simulink library "SNS_Library"  (R2025b)
settings: Solver=VariableStepAuto  StartTime=0.0  StopTime=10.0  RelTol=1e-3
libraries: simulink x3
settings Model: Creator=Ben Bolen  LastModifiedBy=Ben

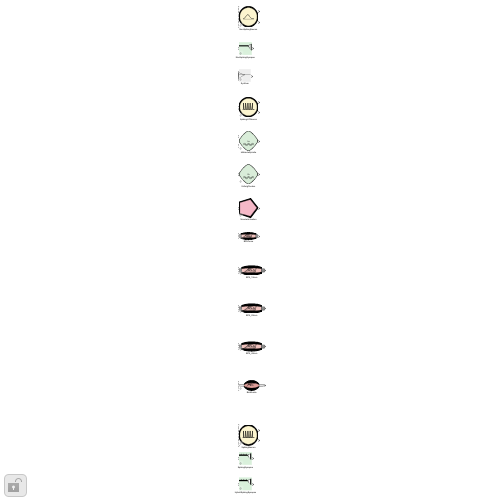
[thumbnail: Simulink's stored preview of the top-level diagram]
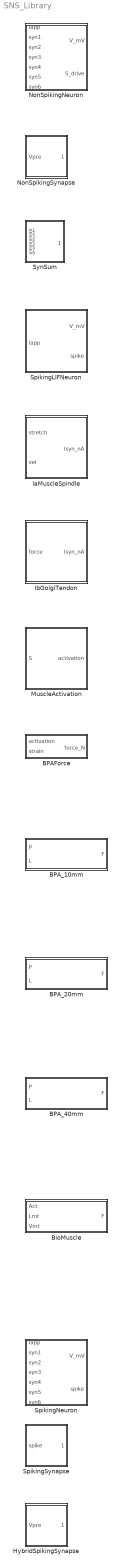
== system SNS_Library ==
  BPAForce : Subsystem  mask(SNS BPA Force Element){Fmax=500, epsMax=0.25}
      mask prompts: Fmax "Max isometric force Fmax (N)"; epsMax "Max contraction strain epsMax (0..1)"
      mask help: Simple BPA (pneumatic artificial muscle) force: F = Fmax*A*max(0, epsMax - strain). Replace with MonoPam/Xi-corrected prediction when available.
      mask Display:
      | patch([-0.7 -0.6708 -0.6417 -0.6125 -0.5833 -0.5542 -0.525 -0.4958 -0.4667 -0.4375 -0.4083 -0.3792 -0.35 -0.3208 -0.2917 -0.2625 -0.2333 -0.2042 -0.175 -0.1458 -0.1167 -0.0875 -0.05833 -0.02917 0 0.02917 0.05833 0.0875 0.1167 0.1458 0.175 0.2042 0.2333 0.2625 0.2917 0.3208 0.35 0.3792 0.4083 0.4375 0.4667 0.4958 0.525 0.5542 0.5833 0.6125 0.6417 0.6708 0.7 0.7 0.6708 0.6417 0.6125 0.5833 0.5542 0.525 0.4958 0.4667 0.4375 0.4083 0.3792 0.35 0.3208 0.2917 0.2625 0.2333 0.2042 0.175 0.1458 0.1167 0.0875 0.05833 0.02917 0 -0.02917 -0.05833 -0.0875 -0.1167 -0.1458 -0.175 -0.2042 -0.2333 -0.2625 -0.2917 -0.3208 -0.35 -0.3792 -0.4083 -0.4375 -0.4667 -0.4958 -0.525 -0.5542 -0.5833 -0.6125 -0.6417 -0.6708 -0.7], [0.395 0.4138 0.4317 0.4489 0.4653 0.4809 0.4956 0.5096 0.5228 0.5352 0.5467 0.5575 0.5675 0.5767 0.5851 0.5927 0.5994 0.6054 0.6106 0.615 0.6186 0.6214 0.6234 0.6246 0.625 0.6246 0.6234 0.6214 0.6186 0.615 0.6106 0.6054 0.5994 0.5927 0.5851 0.5767 0.5675 0.5575 0.5467 0.5352 0.5228 0.5096 0.4956 0.4809 0.4653 0.4489 0.4317 0.4138 0.395 -0.395 -0.4138 -0.4317 -0.4489 -0.4653 -0.4809 -0.4956 -0.5096 -0.5228 -0.5352 -0.5467 -0.5575 -0.5675 -0.5767 -0.5851 -0.5927 -0.5994 -0.6054 -0.6106 -0.615 -0.6186 -0.6214 -0.6234 -0.6246 -0.625 -0.6246 -0.6234 -0.6214 -0.6186 -0.615 -0.6106 -0.6054 -0.5994 -0.5927 -0.5851 -0.5767 -0.5675 -0.5575 -0.5467 -0.5352 -0.5228 -0.5096 -0.4956 -0.4809 -0.4653 -0.4489 -0.4317 -0.4138 -0.395], [0 0 0]);
      | patch([-0.7 -0.6708 -0.6417 -0.6125 -0.5833 -0.5542 -0.525 -0.4958 -0.4667 -0.4375 -0.4083 -0.3792 -0.35 -0.3208 -0.2917 -0.2625 -0.2333 -0.2042 -0.175 -0.1458 -0.1167 -0.0875 -0.05833 -0.02917 0 0.02917 0.05833 0.0875 0.1167 0.1458 0.175 0.2042 0.2333 0.2625 0.2917 0.3208 0.35 0.3792 0.4083 0.4375 0.4667 0.4958 0.525 0.5542 0.5833 0.6125 0.6417 0.6708 0.7 0.7 0.6708 0.6417 0.6125 0.5833 0.5542 0.525 0.4958 0.4667 0.4375 0.4083 0.3792 0.35 0.3208 0.2917 0.2625 0.2333 0.2042 0.175 0.1458 0.1167 0.0875 0.05833 0.02917 0 -0.02917 -0.05833 -0.0875 -0.1167 -0.1458 -0.175 -0.2042 -0.2333 -0.2625 -0.2917 -0.3208 -0.35 -0.3792 -0.4083 -0.4375 -0.4667 -0.4958 -0.525 -0.5542 -0.5833 -0.6125 -0.6417 -0.6708 -0.7], [0.185 0.1944 0.2034 0.212 0.2201 0.2279 0.2353 0.2423 0.2489 0.2551 0.2609 0.2663 0.2712 0.2758 0.28 0.2838 0.2872 0.2902 0.2928 0.295 0.2968 0.2982 0.2992 0.2998 0.3 0.2998 0.2992 0.2982 0.2968 0.295 0.2928 0.2902 0.2872 0.2838 0.28 0.2758 0.2712 0.2663 0.2609 0.2551 0.2489 0.2423 0.2353 0.2279 0.2201 0.212 0.2034 0.1944 0.185 -0.185 -0.1944 -0.2034 -0.212 -0.2201 -0.2279 -0.2353 -0.2423 -0.2489 -0.2551 -0.2609 -0.2663 -0.2712 -0.2758 -0.28 -0.2838 -0.2872 -0.2902 -0.2928 -0.295 -0.2968 -0.2982 -0.2992 -0.2998 -0.3 -0.2998 -0.2992 -0.2982 -0.2968 -0.295 -0.2928 -0.2902 -0.2872 -0.2838 -0.28 -0.2758 -0.2712 -0.2663 -0.2609 -0.2551 -0.2489 -0.2423 -0.2353 -0.2279 -0.2201 -0.212 -0.2034 -0.1944 -0.185], [0.94 0.76 0.74]);
      | color('black');
      | plot([-0.64 -0.1835], [-0.34 0.2456]);
      | plot([-0.64 0.1835], [-0.34 -0.2456]);
      | plot([-0.465 -0.2243], [-0.165 0.2642]);
      | plot([-0.465 0.2243], [-0.165 -0.2642]);
      | plot([-0.29 -0.2522], [0.01 0.27]);
      | plot([-0.29 0.2522], [0.01 -0.27]);
      | plot([-0.115 -0.2672], [0.185 0.2628]);
      | plot([-0.115 0.2672], [0.185 -0.2628]);
      | plot([0.06 -0.2692], [0.36 0.2426]);
      | plot([0.06 0.2692], [0.36 -0.2426]);
      | plot([0.235 -0.2583], [0.535 0.2095]);
      | plot([0.235 0.2583], [0.535 -0.2095]);
      | plot([0.41 -0.2345], [0.66 0.178]);
      | plot([0.41 0.2345], [0.66 -0.178]);
      | patch([0.7 0.9 0.9 0.7], [-0.218 -0.218 0.218 0.218], [0 0 0]);
      | patch([0.7 0.9 0.9 0.7], [-0.2 -0.2 0.2 0.2], [0.55 0.55 0.55]);
      | patch([-0.7 -0.9 -0.9 -0.7], [-0.218 -0.218 0.218 0.218], [0 0 0]);
      | patch([-0.7 -0.9 -0.9 -0.7], [-0.2 -0.2 0.2 0.2], [0.55 0.55 0.55]);
      | disp('BPA');
  BPA_10mm : Subsystem  mask(SNS BPA 10 mm Actuator){Rest=0.20, Kmax=0.165, TendonL=0, FittingL=0}
      mask prompts: Rest "Resting length Rest (m)"; Kmax "Fully-contracted length Kmax (m)"; TendonL "Tendon length (m)"; FittingL "One end-fitting length (m)"
      mask help: Real Festo BPA actuator, 10 mm ID, Ben's equations: F = Fmax*[a0*(exp(-a1*rel)-1) + (P/620)*exp(-a3*rel^2)], rel = contraction/KMAX, contraction = (Rest-(L-TendonL-2*FittingL))/Rest. Zero force for rel>=1 and F<0 (festo4.m). Fmax = maxBPAforce(Rest,620) is baked into the internal gain (edit inside the block to override); Inputs: P [kPa], L [m]. Output: F [N].
      mask Display:
      | patch([-0.7 -0.6708 -0.6417 -0.6125 -0.5833 -0.5542 -0.525 -0.4958 -0.4667 -0.4375 -0.4083 -0.3792 -0.35 -0.3208 -0.2917 -0.2625 -0.2333 -0.2042 -0.175 -0.1458 -0.1167 -0.0875 -0.05833 -0.02917 0 0.02917 0.05833 0.0875 0.1167 0.1458 0.175 0.2042 0.2333 0.2625 0.2917 0.3208 0.35 0.3792 0.4083 0.4375 0.4667 0.4958 0.525 0.5542 0.5833 0.6125 0.6417 0.6708 0.7 0.7 0.6708 0.6417 0.6125 0.5833 0.5542 0.525 0.4958 0.4667 0.4375 0.4083 0.3792 0.35 0.3208 0.2917 0.2625 0.2333 0.2042 0.175 0.1458 0.1167 0.0875 0.05833 0.02917 0 -0.02917 -0.05833 -0.0875 -0.1167 -0.1458 -0.175 -0.2042 -0.2333 -0.2625 -0.2917 -0.3208 -0.35 -0.3792 -0.4083 -0.4375 -0.4667 -0.4958 -0.525 -0.5542 -0.5833 -0.6125 -0.6417 -0.6708 -0.7], [0.395 0.4138 0.4317 0.4489 0.4653 0.4809 0.4956 0.5096 0.5228 0.5352 0.5467 0.5575 0.5675 0.5767 0.5851 0.5927 0.5994 0.6054 0.6106 0.615 0.6186 0.6214 0.6234 0.6246 0.625 0.6246 0.6234 0.6214 0.6186 0.615 0.6106 0.6054 0.5994 0.5927 0.5851 0.5767 0.5675 0.5575 0.5467 0.5352 0.5228 0.5096 0.4956 0.4809 0.4653 0.4489 0.4317 0.4138 0.395 -0.395 -0.4138 -0.4317 -0.4489 -0.4653 -0.4809 -0.4956 -0.5096 -0.5228 -0.5352 -0.5467 -0.5575 -0.5675 -0.5767 -0.5851 -0.5927 -0.5994 -0.6054 -0.6106 -0.615 -0.6186 -0.6214 -0.6234 -0.6246 -0.625 -0.6246 -0.6234 -0.6214 -0.6186 -0.615 -0.6106 -0.6054 -0.5994 -0.5927 -0.5851 -0.5767 -0.5675 -0.5575 -0.5467 -0.5352 -0.5228 -0.5096 -0.4956 -0.4809 -0.4653 -0.4489 -0.4317 -0.4138 -0.395], [0 0 0]);
      | patch([-0.7 -0.6708 -0.6417 -0.6125 -0.5833 -0.5542 -0.525 -0.4958 -0.4667 -0.4375 -0.4083 -0.3792 -0.35 -0.3208 -0.2917 -0.2625 -0.2333 -0.2042 -0.175 -0.1458 -0.1167 -0.0875 -0.05833 -0.02917 0 0.02917 0.05833 0.0875 0.1167 0.1458 0.175 0.2042 0.2333 0.2625 0.2917 0.3208 0.35 0.3792 0.4083 0.4375 0.4667 0.4958 0.525 0.5542 0.5833 0.6125 0.6417 0.6708 0.7 0.7 0.6708 0.6417 0.6125 0.5833 0.5542 0.525 0.4958 0.4667 0.4375 0.4083 0.3792 0.35 0.3208 0.2917 0.2625 0.2333 0.2042 0.175 0.1458 0.1167 0.0875 0.05833 0.02917 0 -0.02917 -0.05833 -0.0875 -0.1167 -0.1458 -0.175 -0.2042 -0.2333 -0.2625 -0.2917 -0.3208 -0.35 -0.3792 -0.4083 -0.4375 -0.4667 -0.4958 -0.525 -0.5542 -0.5833 -0.6125 -0.6417 -0.6708 -0.7], [0.185 0.1944 0.2034 0.212 0.2201 0.2279 0.2353 0.2423 0.2489 0.2551 0.2609 0.2663 0.2712 0.2758 0.28 0.2838 0.2872 0.2902 0.2928 0.295 0.2968 0.2982 0.2992 0.2998 0.3 0.2998 0.2992 0.2982 0.2968 0.295 0.2928 0.2902 0.2872 0.2838 0.28 0.2758 0.2712 0.2663 0.2609 0.2551 0.2489 0.2423 0.2353 0.2279 0.2201 0.212 0.2034 0.1944 0.185 -0.185 -0.1944 -0.2034 -0.212 -0.2201 -0.2279 -0.2353 -0.2423 -0.2489 -0.2551 -0.2609 -0.2663 -0.2712 -0.2758 -0.28 -0.2838 -0.2872 -0.2902 -0.2928 -0.295 -0.2968 -0.2982 -0.2992 -0.2998 -0.3 -0.2998 -0.2992 -0.2982 -0.2968 -0.295 -0.2928 -0.2902 -0.2872 -0.2838 -0.28 -0.2758 -0.2712 -0.2663 -0.2609 -0.2551 -0.2489 -0.2423 -0.2353 -0.2279 -0.2201 -0.212 -0.2034 -0.1944 -0.185], [0.94 0.76 0.74]);
      | color('black');
      | plot([-0.64 -0.1835], [-0.34 0.2456]);
      | plot([-0.64 0.1835], [-0.34 -0.2456]);
      | plot([-0.465 -0.2243], [-0.165 0.2642]);
      | plot([-0.465 0.2243], [-0.165 -0.2642]);
      | plot([-0.29 -0.2522], [0.01 0.27]);
      | plot([-0.29 0.2522], [0.01 -0.27]);
      | plot([-0.115 -0.2672], [0.185 0.2628]);
      | plot([-0.115 0.2672], [0.185 -0.2628]);
      | plot([0.06 -0.2692], [0.36 0.2426]);
      | plot([0.06 0.2692], [0.36 -0.2426]);
      | plot([0.235 -0.2583], [0.535 0.2095]);
      | plot([0.235 0.2583], [0.535 -0.2095]);
      | plot([0.41 -0.2345], [0.66 0.178]);
      | plot([0.41 0.2345], [0.66 -0.178]);
      | patch([0.7 0.9 0.9 0.7], [-0.218 -0.218 0.218 0.218], [0 0 0]);
      | patch([0.7 0.9 0.9 0.7], [-0.2 -0.2 0.2 0.2], [0.55 0.55 0.55]);
      | patch([-0.7 -0.9 -0.9 -0.7], [-0.218 -0.218 0.218 0.218], [0 0 0]);
      | patch([-0.7 -0.9 -0.9 -0.7], [-0.2 -0.2 0.2 0.2], [0.55 0.55 0.55]);
      | disp('BPA 10');
  BPA_20mm : Subsystem  mask(SNS BPA 20 mm Actuator){Rest=0.20, Kmax=0.165, TendonL=0, FittingL=0}
      mask prompts: Rest "Resting length Rest (m)"; Kmax "Fully-contracted length Kmax (m)"; TendonL "Tendon length (m)"; FittingL "One end-fitting length (m)"
      mask help: Real Festo BPA actuator, 20 mm ID, Ben's equations: F = Fmax*[a0*(exp(-a1*rel)-1) + (P/620)*exp(-a3*rel^2)], rel = contraction/KMAX, contraction = (Rest-(L-TendonL-2*FittingL))/Rest. Zero force for rel>=1 and F<0 (festo4.m). Fmax = maxBPAforce(Rest,620) is baked into the internal gain (edit inside the block to override); Inputs: P [kPa], L [m]. Output: F [N].
      mask Display:
      | patch([-0.7 -0.6708 -0.6417 -0.6125 -0.5833 -0.5542 -0.525 -0.4958 -0.4667 -0.4375 -0.4083 -0.3792 -0.35 -0.3208 -0.2917 -0.2625 -0.2333 -0.2042 -0.175 -0.1458 -0.1167 -0.0875 -0.05833 -0.02917 0 0.02917 0.05833 0.0875 0.1167 0.1458 0.175 0.2042 0.2333 0.2625 0.2917 0.3208 0.35 0.3792 0.4083 0.4375 0.4667 0.4958 0.525 0.5542 0.5833 0.6125 0.6417 0.6708 0.7 0.7 0.6708 0.6417 0.6125 0.5833 0.5542 0.525 0.4958 0.4667 0.4375 0.4083 0.3792 0.35 0.3208 0.2917 0.2625 0.2333 0.2042 0.175 0.1458 0.1167 0.0875 0.05833 0.02917 0 -0.02917 -0.05833 -0.0875 -0.1167 -0.1458 -0.175 -0.2042 -0.2333 -0.2625 -0.2917 -0.3208 -0.35 -0.3792 -0.4083 -0.4375 -0.4667 -0.4958 -0.525 -0.5542 -0.5833 -0.6125 -0.6417 -0.6708 -0.7], [0.395 0.4138 0.4317 0.4489 0.4653 0.4809 0.4956 0.5096 0.5228 0.5352 0.5467 0.5575 0.5675 0.5767 0.5851 0.5927 0.5994 0.6054 0.6106 0.615 0.6186 0.6214 0.6234 0.6246 0.625 0.6246 0.6234 0.6214 0.6186 0.615 0.6106 0.6054 0.5994 0.5927 0.5851 0.5767 0.5675 0.5575 0.5467 0.5352 0.5228 0.5096 0.4956 0.4809 0.4653 0.4489 0.4317 0.4138 0.395 -0.395 -0.4138 -0.4317 -0.4489 -0.4653 -0.4809 -0.4956 -0.5096 -0.5228 -0.5352 -0.5467 -0.5575 -0.5675 -0.5767 -0.5851 -0.5927 -0.5994 -0.6054 -0.6106 -0.615 -0.6186 -0.6214 -0.6234 -0.6246 -0.625 -0.6246 -0.6234 -0.6214 -0.6186 -0.615 -0.6106 -0.6054 -0.5994 -0.5927 -0.5851 -0.5767 -0.5675 -0.5575 -0.5467 -0.5352 -0.5228 -0.5096 -0.4956 -0.4809 -0.4653 -0.4489 -0.4317 -0.4138 -0.395], [0 0 0]);
      | patch([-0.7 -0.6708 -0.6417 -0.6125 -0.5833 -0.5542 -0.525 -0.4958 -0.4667 -0.4375 -0.4083 -0.3792 -0.35 -0.3208 -0.2917 -0.2625 -0.2333 -0.2042 -0.175 -0.1458 -0.1167 -0.0875 -0.05833 -0.02917 0 0.02917 0.05833 0.0875 0.1167 0.1458 0.175 0.2042 0.2333 0.2625 0.2917 0.3208 0.35 0.3792 0.4083 0.4375 0.4667 0.4958 0.525 0.5542 0.5833 0.6125 0.6417 0.6708 0.7 0.7 0.6708 0.6417 0.6125 0.5833 0.5542 0.525 0.4958 0.4667 0.4375 0.4083 0.3792 0.35 0.3208 0.2917 0.2625 0.2333 0.2042 0.175 0.1458 0.1167 0.0875 0.05833 0.02917 0 -0.02917 -0.05833 -0.0875 -0.1167 -0.1458 -0.175 -0.2042 -0.2333 -0.2625 -0.2917 -0.3208 -0.35 -0.3792 -0.4083 -0.4375 -0.4667 -0.4958 -0.525 -0.5542 -0.5833 -0.6125 -0.6417 -0.6708 -0.7], [0.185 0.1944 0.2034 0.212 0.2201 0.2279 0.2353 0.2423 0.2489 0.2551 0.2609 0.2663 0.2712 0.2758 0.28 0.2838 0.2872 0.2902 0.2928 0.295 0.2968 0.2982 0.2992 0.2998 0.3 0.2998 0.2992 0.2982 0.2968 0.295 0.2928 0.2902 0.2872 0.2838 0.28 0.2758 0.2712 0.2663 0.2609 0.2551 0.2489 0.2423 0.2353 0.2279 0.2201 0.212 0.2034 0.1944 0.185 -0.185 -0.1944 -0.2034 -0.212 -0.2201 -0.2279 -0.2353 -0.2423 -0.2489 -0.2551 -0.2609 -0.2663 -0.2712 -0.2758 -0.28 -0.2838 -0.2872 -0.2902 -0.2928 -0.295 -0.2968 -0.2982 -0.2992 -0.2998 -0.3 -0.2998 -0.2992 -0.2982 -0.2968 -0.295 -0.2928 -0.2902 -0.2872 -0.2838 -0.28 -0.2758 -0.2712 -0.2663 -0.2609 -0.2551 -0.2489 -0.2423 -0.2353 -0.2279 -0.2201 -0.212 -0.2034 -0.1944 -0.185], [0.94 0.76 0.74]);
      | color('black');
      | plot([-0.64 -0.1835], [-0.34 0.2456]);
      | plot([-0.64 0.1835], [-0.34 -0.2456]);
      | plot([-0.465 -0.2243], [-0.165 0.2642]);
      | plot([-0.465 0.2243], [-0.165 -0.2642]);
      | plot([-0.29 -0.2522], [0.01 0.27]);
      | plot([-0.29 0.2522], [0.01 -0.27]);
      | plot([-0.115 -0.2672], [0.185 0.2628]);
      | plot([-0.115 0.2672], [0.185 -0.2628]);
      | plot([0.06 -0.2692], [0.36 0.2426]);
      | plot([0.06 0.2692], [0.36 -0.2426]);
      | plot([0.235 -0.2583], [0.535 0.2095]);
      | plot([0.235 0.2583], [0.535 -0.2095]);
      | plot([0.41 -0.2345], [0.66 0.178]);
      | plot([0.41 0.2345], [0.66 -0.178]);
      | patch([0.7 0.9 0.9 0.7], [-0.218 -0.218 0.218 0.218], [0 0 0]);
      | patch([0.7 0.9 0.9 0.7], [-0.2 -0.2 0.2 0.2], [0.55 0.55 0.55]);
      | patch([-0.7 -0.9 -0.9 -0.7], [-0.218 -0.218 0.218 0.218], [0 0 0]);
      | patch([-0.7 -0.9 -0.9 -0.7], [-0.2 -0.2 0.2 0.2], [0.55 0.55 0.55]);
      | disp('BPA 20');
  BPA_40mm : Subsystem  mask(SNS BPA 40 mm Actuator){Rest=0.20, Kmax=0.165, TendonL=0, FittingL=0}
      mask prompts: Rest "Resting length Rest (m)"; Kmax "Fully-contracted length Kmax (m)"; TendonL "Tendon length (m)"; FittingL "One end-fitting length (m)"
      mask help: Real Festo BPA actuator, 40 mm ID, Ben's equations: F = Fmax*[a0*(exp(-a1*rel)-1) + (P/620)*exp(-a3*rel^2)], rel = contraction/KMAX, contraction = (Rest-(L-TendonL-2*FittingL))/Rest. Zero force for rel>=1 and F<0 (festo4.m). Fmax = maxBPAforce(Rest,620) is baked into the internal gain (edit inside the block to override); Inputs: P [kPa], L [m]. Output: F [N].
      mask Display:
      | patch([-0.7 -0.6708 -0.6417 -0.6125 -0.5833 -0.5542 -0.525 -0.4958 -0.4667 -0.4375 -0.4083 -0.3792 -0.35 -0.3208 -0.2917 -0.2625 -0.2333 -0.2042 -0.175 -0.1458 -0.1167 -0.0875 -0.05833 -0.02917 0 0.02917 0.05833 0.0875 0.1167 0.1458 0.175 0.2042 0.2333 0.2625 0.2917 0.3208 0.35 0.3792 0.4083 0.4375 0.4667 0.4958 0.525 0.5542 0.5833 0.6125 0.6417 0.6708 0.7 0.7 0.6708 0.6417 0.6125 0.5833 0.5542 0.525 0.4958 0.4667 0.4375 0.4083 0.3792 0.35 0.3208 0.2917 0.2625 0.2333 0.2042 0.175 0.1458 0.1167 0.0875 0.05833 0.02917 0 -0.02917 -0.05833 -0.0875 -0.1167 -0.1458 -0.175 -0.2042 -0.2333 -0.2625 -0.2917 -0.3208 -0.35 -0.3792 -0.4083 -0.4375 -0.4667 -0.4958 -0.525 -0.5542 -0.5833 -0.6125 -0.6417 -0.6708 -0.7], [0.395 0.4138 0.4317 0.4489 0.4653 0.4809 0.4956 0.5096 0.5228 0.5352 0.5467 0.5575 0.5675 0.5767 0.5851 0.5927 0.5994 0.6054 0.6106 0.615 0.6186 0.6214 0.6234 0.6246 0.625 0.6246 0.6234 0.6214 0.6186 0.615 0.6106 0.6054 0.5994 0.5927 0.5851 0.5767 0.5675 0.5575 0.5467 0.5352 0.5228 0.5096 0.4956 0.4809 0.4653 0.4489 0.4317 0.4138 0.395 -0.395 -0.4138 -0.4317 -0.4489 -0.4653 -0.4809 -0.4956 -0.5096 -0.5228 -0.5352 -0.5467 -0.5575 -0.5675 -0.5767 -0.5851 -0.5927 -0.5994 -0.6054 -0.6106 -0.615 -0.6186 -0.6214 -0.6234 -0.6246 -0.625 -0.6246 -0.6234 -0.6214 -0.6186 -0.615 -0.6106 -0.6054 -0.5994 -0.5927 -0.5851 -0.5767 -0.5675 -0.5575 -0.5467 -0.5352 -0.5228 -0.5096 -0.4956 -0.4809 -0.4653 -0.4489 -0.4317 -0.4138 -0.395], [0 0 0]);
      | patch([-0.7 -0.6708 -0.6417 -0.6125 -0.5833 -0.5542 -0.525 -0.4958 -0.4667 -0.4375 -0.4083 -0.3792 -0.35 -0.3208 -0.2917 -0.2625 -0.2333 -0.2042 -0.175 -0.1458 -0.1167 -0.0875 -0.05833 -0.02917 0 0.02917 0.05833 0.0875 0.1167 0.1458 0.175 0.2042 0.2333 0.2625 0.2917 0.3208 0.35 0.3792 0.4083 0.4375 0.4667 0.4958 0.525 0.5542 0.5833 0.6125 0.6417 0.6708 0.7 0.7 0.6708 0.6417 0.6125 0.5833 0.5542 0.525 0.4958 0.4667 0.4375 0.4083 0.3792 0.35 0.3208 0.2917 0.2625 0.2333 0.2042 0.175 0.1458 0.1167 0.0875 0.05833 0.02917 0 -0.02917 -0.05833 -0.0875 -0.1167 -0.1458 -0.175 -0.2042 -0.2333 -0.2625 -0.2917 -0.3208 -0.35 -0.3792 -0.4083 -0.4375 -0.4667 -0.4958 -0.525 -0.5542 -0.5833 -0.6125 -0.6417 -0.6708 -0.7], [0.185 0.1944 0.2034 0.212 0.2201 0.2279 0.2353 0.2423 0.2489 0.2551 0.2609 0.2663 0.2712 0.2758 0.28 0.2838 0.2872 0.2902 0.2928 0.295 0.2968 0.2982 0.2992 0.2998 0.3 0.2998 0.2992 0.2982 0.2968 0.295 0.2928 0.2902 0.2872 0.2838 0.28 0.2758 0.2712 0.2663 0.2609 0.2551 0.2489 0.2423 0.2353 0.2279 0.2201 0.212 0.2034 0.1944 0.185 -0.185 -0.1944 -0.2034 -0.212 -0.2201 -0.2279 -0.2353 -0.2423 -0.2489 -0.2551 -0.2609 -0.2663 -0.2712 -0.2758 -0.28 -0.2838 -0.2872 -0.2902 -0.2928 -0.295 -0.2968 -0.2982 -0.2992 -0.2998 -0.3 -0.2998 -0.2992 -0.2982 -0.2968 -0.295 -0.2928 -0.2902 -0.2872 -0.2838 -0.28 -0.2758 -0.2712 -0.2663 -0.2609 -0.2551 -0.2489 -0.2423 -0.2353 -0.2279 -0.2201 -0.212 -0.2034 -0.1944 -0.185], [0.94 0.76 0.74]);
      | color('black');
      | plot([-0.64 -0.1835], [-0.34 0.2456]);
      | plot([-0.64 0.1835], [-0.34 -0.2456]);
      | plot([-0.465 -0.2243], [-0.165 0.2642]);
      | plot([-0.465 0.2243], [-0.165 -0.2642]);
      | plot([-0.29 -0.2522], [0.01 0.27]);
      | plot([-0.29 0.2522], [0.01 -0.27]);
      | plot([-0.115 -0.2672], [0.185 0.2628]);
      | plot([-0.115 0.2672], [0.185 -0.2628]);
      | plot([0.06 -0.2692], [0.36 0.2426]);
      | plot([0.06 0.2692], [0.36 -0.2426]);
      | plot([0.235 -0.2583], [0.535 0.2095]);
      | plot([0.235 0.2583], [0.535 -0.2095]);
      | plot([0.41 -0.2345], [0.66 0.178]);
      | plot([0.41 0.2345], [0.66 -0.178]);
      | patch([0.7 0.9 0.9 0.7], [-0.218 -0.218 0.218 0.218], [0 0 0]);
      | patch([0.7 0.9 0.9 0.7], [-0.2 -0.2 0.2 0.2], [0.55 0.55 0.55]);
      | patch([-0.7 -0.9 -0.9 -0.7], [-0.218 -0.218 0.218 0.218], [0 0 0]);
      | patch([-0.7 -0.9 -0.9 -0.7], [-0.2 -0.2 0.2 0.2], [0.55 0.55 0.55]);
      | disp('BPA 40');
  BioMuscle : Subsystem  mask(SNS Biological Muscle (Thelen-style)){Fmax=1000, l_opt=0.10, l_slack=0.05, alpha=0, v_max=10, A_hill=0.25, kpe=4, e_pas=0.6}
      mask prompts: Fmax "Max isometric force Fmax (N)"; l_opt "Optimal fiber length l_opt (m)"; l_slack "Tendon slack length (m)"; alpha "Pennation angle (deg)"; v_max "Max shortening velocity (l_opt/s)"; A_hill "Hill curvature A (a/Fmax)"; kpe "Passive FL exponent kpe"; e_pas "Passive FL strain at Fmax e_pas"
      mask help: OpenSim Thelen2003-style Hill-type biological muscle, rigid tendon: F = Fmax*(Act*fl(lambda)*fv(v) + fpas(lambda))*cos(alpha). Active FL = exp(-(lambda-1)^2/0.45); Hill force-velocity (A=0.25, v_max in l_opt/s); exponential passive FL (kpe, e_pas); fiber length = (Lmt-l_slack)/cos(alpha). Inputs: Act [0..1], Lmt [m], Vmt [m/s]. Output: F [N].
      mask Display:
      | patch([-0.58 -0.5558 -0.5317 -0.5075 -0.4833 -0.4592 -0.435 -0.4108 -0.3867 -0.3625 -0.3383 -0.3142 -0.29 -0.2658 -0.2417 -0.2175 -0.1933 -0.1692 -0.145 -0.1208 -0.09667 -0.0725 -0.04833 -0.02417 0 0.02417 0.04833 0.0725 0.09667 0.1208 0.145 0.1692 0.1933 0.2175 0.2417 0.2658 0.29 0.3142 0.3383 0.3625 0.3867 0.4108 0.435 0.4592 0.4833 0.5075 0.5317 0.5558 0.58 0.58 0.5558 0.5317 0.5075 0.4833 0.4592 0.435 0.4108 0.3867 0.3625 0.3383 0.3142 0.29 0.2658 0.2417 0.2175 0.1933 0.1692 0.145 0.1208 0.09667 0.0725 0.04833 0.02417 0 -0.02417 -0.04833 -0.0725 -0.09667 -0.1208 -0.145 -0.1692 -0.1933 -0.2175 -0.2417 -0.2658 -0.29 -0.3142 -0.3383 -0.3625 -0.3867 -0.4108 -0.435 -0.4592 -0.4833 -0.5075 -0.5317 -0.5558 -0.58], [0.022 0.1323 0.2009 0.2577 0.3073 0.3516 0.3915 0.4277 0.4608 0.491 0.5186 0.5438 0.5667 0.5874 0.606 0.6227 0.6375 0.6505 0.6616 0.6709 0.6785 0.6844 0.6886 0.6912 0.692 0.6912 0.6886 0.6844 0.6785 0.6709 0.6616 0.6505 0.6375 0.6227 0.606 0.5874 0.5667 0.5438 0.5186 0.491 0.4608 0.4277 0.3915 0.3516 0.3073 0.2577 0.2009 0.1323 0.022 0.022 -0.1323 -0.2009 -0.2577 -0.3073 -0.3516 -0.3915 -0.4277 -0.4608 -0.491 -0.5186 -0.5438 -0.5667 -0.5874 -0.606 -0.6227 -0.6375 -0.6505 -0.6616 -0.6709 -0.6785 -0.6844 -0.6886 -0.6912 -0.692 -0.6912 -0.6886 -0.6844 -0.6785 -0.6709 -0.6616 -0.6505 -0.6375 -0.6227 -0.606 -0.5874 -0.5667 -0.5438 -0.5186 -0.491 -0.4608 -0.4277 -0.3915 -0.3516 -0.3073 -0.2577 -0.2009 -0.1323 0.022], [0 0 0]);
      | patch([-0.58 -0.5558 -0.5317 -0.5075 -0.4833 -0.4592 -0.435 -0.4108 -0.3867 -0.3625 -0.3383 -0.3142 -0.29 -0.2658 -0.2417 -0.2175 -0.1933 -0.1692 -0.145 -0.1208 -0.09667 -0.0725 -0.04833 -0.02417 0 0.02417 0.04833 0.0725 0.09667 0.1208 0.145 0.1692 0.1933 0.2175 0.2417 0.2658 0.29 0.3142 0.3383 0.3625 0.3867 0.4108 0.435 0.4592 0.4833 0.5075 0.5317 0.5558 0.58 0.58 0.5558 0.5317 0.5075 0.4833 0.4592 0.435 0.4108 0.3867 0.3625 0.3383 0.3142 0.29 0.2658 0.2417 0.2175 0.1933 0.1692 0.145 0.1208 0.09667 0.0725 0.04833 0.02417 0 -0.02417 -0.04833 -0.0725 -0.09667 -0.1208 -0.145 -0.1692 -0.1933 -0.2175 -0.2417 -0.2658 -0.29 -0.3142 -0.3383 -0.3625 -0.3867 -0.4108 -0.435 -0.4592 -0.4833 -0.5075 -0.5317 -0.5558 -0.58], [0 0.05514 0.08943 0.1179 0.1427 0.1648 0.1847 0.2029 0.2194 0.2345 0.2483 0.2609 0.2723 0.2827 0.292 0.3004 0.3078 0.3142 0.3198 0.3245 0.3283 0.3312 0.3333 0.3346 0.335 0.3346 0.3333 0.3312 0.3283 0.3245 0.3198 0.3142 0.3078 0.3004 0.292 0.2827 0.2723 0.2609 0.2483 0.2345 0.2194 0.2029 0.1847 0.1648 0.1427 0.1179 0.08943 0.05514 0 -0 -0.05514 -0.08943 -0.1179 -0.1427 -0.1648 -0.1847 -0.2029 -0.2194 -0.2345 -0.2483 -0.2609 -0.2723 -0.2827 -0.292 -0.3004 -0.3078 -0.3142 -0.3198 -0.3245 -0.3283 -0.3312 -0.3333 -0.3346 -0.335 -0.3346 -0.3333 -0.3312 -0.3283 -0.3245 -0.3198 -0.3142 -0.3078 -0.3004 -0.292 -0.2827 -0.2723 -0.2609 -0.2483 -0.2345 -0.2194 -0.2029 -0.1847 -0.1648 -0.1427 -0.1179 -0.08943 -0.05514 -0], [0.87 0.62 0.6]);
      | color('black');
      | plot([-0.46 -0.1476], [-0.2855 0.2469]);
      | plot([-0.305 -0.2388], [-0.02282 0.3012]);
      | plot([-0.15 -0.2868], [0.1889 0.2781]);
      | plot([0.005 -0.3015], [0.3612 0.2117]);
      | plot([0.16 -0.2848], [0.4965 0.1166]);
      | plot([0.315 -0.2344], [0.52 0.09333]);
      | plot([0.47 -0.1396], [0.52 0.09333]);
      | patch([0.58 0.95 0.95 0.58], [-0.148 -0.068 0.068 0.148], [0 0 0]);
      | patch([0.58 0.95 0.95 0.58], [-0.13 -0.05 0.05 0.13], [0.88 0.88 0.88]);
      | patch([-0.58 -0.95 -0.95 -0.58], [-0.148 -0.068 0.068 0.148], [0 0 0]);
      | patch([-0.58 -0.95 -0.95 -0.58], [-0.13 -0.05 0.05 0.13], [0.88 0.88 0.88]);
      | disp('BIO');
  HybridSpikingSynapse : Subsystem  mask(SNS Hybrid Spiking Synapse){gmax=1, ginc=1, tau_syn=20, Esyn=0, ThrPre=-45}
      mask prompts: gmax "Max conductance gmax (uS)"; ginc "Conductance increment per spike (uS)"; tau_syn "Decay time constant tau_syn (ms)"; Esyn "Reversal potential Esyn (mV). >=0 excit, <0 inhib"; ThrPre "Spike-detection threshold ThrPre (mV)"
      mask help: HYBRID spiking-to-non-spiking synapse (toolbox Tutorials 3/5/9 pattern: spikes above, analog voltages into the plant). Input: presynaptic membrane potential Vpre [mV] from ANY neuron (spiking or not) — the synapse detects the spike itself: rising edge of (Vpre >= ThrPre). Conductance: exponential decay with tau_syn; on each detected spike g <- min(gmax, g + ginc). Output [g; g*Esyn] connects to the syn1..syn6 port of a NON-SPIKING (or spiking) postsynaptic neuron. CHOOSING ThrPre (AnimatLab semantics): it must sit BETWEEN the presynaptic Vrest and Vth, comfortably BELOW Vth (a spiking presynaptic cell RESETS at threshold, so its V output never renders values >= Vth — ThrPre = Vth fires nothing; ThrPre ~ 0.9*Vth keys the g jump ~1 ms before the true spike).
      mask Display:
      | es_ = NaN;
      | try
      |     tmp_ = Esyn;
      |     if ischar(tmp_) || isstring(tmp_), tmp_ = eval(tmp_); end
      |     es_ = tmp_;
      | catch
      | end
      | if isnan(es_)
      |     patch([-1 1 1 -1], [-1 -1 1 1], [0.9 0.9 0.9]);
      |     disp('E?');
      | elseif es_ < 0
      |     patch([-1 1 1 -1], [-1 -1 1 1], [0.97 0.86 0.85]);
      |     patch([-1 0.58 0.58 -1], [0.42 0.42 0.58 0.58], [0 0 0]);
      |     t_ = linspace(0, 2*pi, 73);
      |     patch(0.18*cos(t_) + 0.72, 0.50*sin(t_), [0 0 0]);
      |     color('black');
      |     plot([-1 -0.75 -0.65 -0.55 -0.35 -0.25 -0.15 0.05 0.15 0.25 0.45 0.55 0.58], [0.50 0.50 0.72 0.50 0.50 0.72 0.50 0.50 0.72 0.50 0.50 0.50 0.50]);
      | else
      |     patch([-1 1 1 -1], [-1 -1 1 1], [0.85 0.94 0.86]);
      |     patch([-1 0.30 0.30 -1], [0.42 0.42 0.58 0.58], [0 0 0]);
      |     patch([0.30 0.90 0.90], [0.50 0.80 -0.20], [0 0 0]);
      |     patch([0.44 0.76 0.76], [0.50 0.70 -0.10], [1 1 1]);
      |     color('black');
      |     plot([-1 -0.75 -0.65 -0.55 -0.35 -0.25 -0.15 0.05 0.15 0.25 0.30], [0.50 0.50 0.72 0.50 0.50 0.72 0.50 0.50 0.72 0.50 0.50]);
      | end
  IaMuscleSpindle : Subsystem  mask(SNS Ia Muscle Spindle Afferent){Imax=10, Wl=6, Wv=8}
      mask prompts: Imax "Peak current Imax (nA)"; Wl "Length weight Wl (nA)"; Wv "Velocity weight Wv (nA)"
      mask help: Ia spindle afferent: Isyn = clip(Wl*stretch + Wv*velocity, 0, Imax) [nA]. Inputs are normalized (0..1) length and velocity signals. Icon: spindle-shaped capsule.
      mask Display:
      | x_ = linspace(-1, 1, 41);
      | w_ = 0.58*(1 - abs(x_).^1.5);
      | patch([x_ fliplr(x_)], [w_ -fliplr(w_)], [0 0 0]);
      | x2_ = 0.93*x_;
      | w2_ = 0.58*(1 - abs(x2_).^1.5);
      | patch([x2_ fliplr(x2_)], [w2_ -fliplr(w2_)], [0.85 0.93 0.85]);
      | color('black');
      | plot(linspace(-0.55, 0.55, 27), 0.05*sin(linspace(0, 5*pi, 27)) - 0.24);
      | plot(linspace(-0.55, 0.55, 27), 0.05*sin(linspace(0, 5*pi, 27)) - 0.24 + 0.06);
      | disp('Ia');
  IbGolgiTendon : Subsystem  mask(SNS Ib Golgi Tendon Afferent){Imax=10, Kf=10}
      mask prompts: Imax "Peak current Imax (nA)"; Kf "Force weight Kf (nA)"
      mask help: Ib Golgi tendon organ afferent: Isyn = clip(Kf*forceNorm, 0, Imax) [nA]. Input is normalized force (0..1). Icon: capsule with braided collagen strands.
      mask Display:
      | x_ = linspace(-1, 1, 41);
      | w_ = 0.58*(1 - abs(x_).^1.5);
      | patch([x_ fliplr(x_)], [w_ -fliplr(w_)], [0 0 0]);
      | x2_ = 0.93*x_;
      | w2_ = 0.58*(1 - abs(x2_).^1.5);
      | patch([x2_ fliplr(x2_)], [w2_ -fliplr(w2_)], [0.85 0.93 0.85]);
      | color('black');
      | plot(linspace(-0.55, 0.55, 27), 0.05*sin(linspace(0, 5*pi, 27)) - 0.24);
      | plot(linspace(-0.55, 0.55, 27), 0.05*sin(linspace(0, 5*pi, 27)) - 0.24 + 0.06);
      | disp('Ib');
  MuscleActivation : Subsystem  mask(SNS Muscle Activation){tauAct=50, A0=0}
      mask prompts: tauAct "Activation time constant tauAct (ms)"; A0 "Initial activation A(0) [0..1]"
      mask help: First-order activation dynamics: tauAct*dA/dt = (S - A). Maps motoneuron drive S(V) [0..1] to muscle activation A [0..1]. A0 = initial activation (set it to the steady hold activation so a model starts settled, with no startup transient).
      mask Display:
      | patch(0.95*cos([0      1.2566      2.5133      3.7699      5.0265]), 0.95*sin([0      1.2566      2.5133      3.7699      5.0265]), [0 0 0]);
      | patch(0.82*cos([0      1.2566      2.5133      3.7699      5.0265]), 0.82*sin([0      1.2566      2.5133      3.7699      5.0265]), [0.96 0.72 0.78]);
  NonSpikingNeuron : Subsystem  mask(SNS NonSpiking Neuron){Vrest=-52, Gm=0.1, Cm=5, Thr=-55, Slope=1}
      mask prompts: Vrest "Resting potential Vrest (mV)"; Gm "Membrane conductance Gm (uS)"; Cm "Membrane capacitance Cm (nF)"; Thr "Saturation threshold Thr (mV)"; Slope "Saturation slope (1/mV)"
      mask help: Non-spiking leaky integrate-and-fire neuron (RC membrane) with INTERNAL synaptic summation. Port 1 (Iapp): injected current [nA] — descending drive or afferent currents (a vector input is summed element-wise). Ports syn1..syn6: synaptic inputs from NonSpikingSynapse blocks ([g; g*Esyn]); each synapse connects to the NEXT FREE syn port, unconnected ports count as zero (leave them empty). Cm*dV/dt = Gm*(Vrest-V) + Iapp + sum(g*Esyn) - V*sum(g). Outputs: membrane potential V [mV] and normalized drive S(V) [0..1]. Conventions: Animatlab / sns_toolbox (Szczecinski et al. 2017).
      mask Display:
      | t_ = linspace(0, 2*pi, 73);
      | patch(0.95*cos(t_), 0.95*sin(t_), [0 0 0]);
      | patch(0.84*cos(t_), 0.84*sin(t_), [0.99 0.96 0.81]);
      | x_ = linspace(-0.55, 0.55, 61);
      | y_ = -0.20 + 0.40*exp(-((x_+0.08)/0.26).^2);
      | color('black');
      | plot(x_, y_);
      | plot([-0.55 0.55], [-0.20 -0.20]);
  NonSpikingSynapse : Subsystem  mask(SNS NonSpiking Synapse){gmax=1, Esyn=0, ThrPre=-55, SlopePre=1}
      mask prompts: gmax "Max conductance gmax (uS)"; Esyn "Reversal potential Esyn (mV). >=0 excit, <0 inhib"; ThrPre "Pre saturation threshold ThrPre (mV)"; SlopePre "Pre saturation slope SlopePre (1/mV)"
      mask help: Non-spiking chemical synapse, ONE input -> ONE output. Input: presynaptic membrane potential Vpre [mV]. Output: 2-wide synaptic signal [g; g*Esyn] that connects to a NonSpikingSynapse input port (syn1..syn6) of the POSTSYNAPTIC NonSpikingNeuron — place the synapse next to the neuron it synapses onto. g = gmax*Sat(Vpre), Sat = clip((Vpre-ThrPre)/SlopePre, 0, 1); the neuron forms Isyn = sum(g*Esyn) - Vpost*sum(g). Esyn >= 0 mV -> EXCITATORY (icon: white triangle); Esyn < 0 mV -> INHIBITORY (icon: solid black circle). Diagram language: Szczecinski et al. 2017 Fig. 2.
      mask Display:
      | es_ = NaN;
      | try
      |     tmp_ = Esyn;
      |     if ischar(tmp_) || isstring(tmp_), tmp_ = eval(tmp_); end
      |     es_ = tmp_;
      | catch
      | end
      | if isnan(es_)
      |     patch([-1 1 1 -1], [-1 -1 1 1], [0.9 0.9 0.9]);
      |     disp('E?');
      | elseif es_ < 0
      |     patch([-1 1 1 -1], [-1 -1 1 1], [0.97 0.86 0.85]);
      |     patch([-1 0.70 0.70 -1], [0.34 0.34 0.48 0.48], [0 0 0]);
      |     t_ = linspace(0, 2*pi, 73);
      |     patch(0.20*cos(t_) + 0.76, 0.41*sin(t_), [0 0 0]);
      | else
      |     patch([-1 1 1 -1], [-1 -1 1 1], [0.85 0.94 0.86]);
      |     patch([-1 0.42 0.42 -1], [0.34 0.34 0.48 0.48], [0 0 0]);
      |     patch([0.42 0.98 0.98], [0.41 0.72 -0.30], [0 0 0]);
      |     patch([0.55 0.86 0.86], [0.41 0.62 -0.18], [1 1 1]);
      | end
  SpikingLIFNeuron : Subsystem  mask(SNS Spiking LIF Neuron){Vrest=-60, Vth=-50, Rm=10, tau=20}
      mask prompts: Vrest "Resting potential Vrest (mV)"; Vth "Spike threshold Vth (mV)"; Rm "Membrane resistance Rm (MOhm)"; tau "Membrane time constant tau (ms)"
      mask help: Spiking leaky integrate-and-fire neuron: tau*dV/dt = (Vrest-V) + Rm*Iapp; V>=Vth -> output spike flag and membrane resets to Vrest. Input: injected current Iapp [nA] (vector inputs are summed element-wise).
      mask Display:
      | t_ = linspace(0, 2*pi, 73);
      | patch(0.95*cos(t_), 0.95*sin(t_), [0 0 0]);
      | patch(0.84*cos(t_), 0.84*sin(t_), [0.99 0.96 0.81]);
      | xs_ = [-0.58 -0.54 -0.50 -0.46 -0.36 -0.32 -0.28 -0.24 -0.14 -0.10 -0.06 -0.02 0.08 0.12 0.16 0.20 0.30 0.34 0.38 0.42 0.52 0.58];
      | ys_ = [-0.22 -0.22 0.40 -0.22 -0.22 -0.22 0.40 -0.22 -0.22 -0.22 0.40 -0.22 -0.22 -0.22 0.40 -0.22 -0.22 -0.22 0.40 -0.22 -0.22 -0.22];
      | color('black');
      | plot(xs_, ys_);
      | plot(xs_+0.012, ys_);
      | plot(xs_-0.012, ys_);
  SpikingNeuron : Subsystem  mask(SNS Spiking Neuron){Vrest=-52, Vth=-45, Vreset=-60, Gm=0.1, Cm=5}
      mask prompts: Vrest "Resting potential Vrest (mV)"; Vth "Spike threshold Vth (mV)"; Vreset "Reset (and initial) potential Vreset (mV)"; Gm "Membrane conductance Gm (uS)"; Cm "Membrane capacitance Cm (nF)"
      mask help: Spiking leaky integrate-and-fire neuron with INTERNAL synaptic summation (toolbox SpikingNeuron, fixed-threshold variant). Between spikes the membrane is the same RC circuit as NonSpikingNeuron: Cm*dV/dt = Gm*(Vrest-V) + Iapp + sum(g*Esyn) - V*sum(g). When V >= Vth the spike output goes 1 (one-step pulse) and V resets to Vreset (membrane starts at Vreset). Ports: 1 = Iapp [nA]; syn1..syn6 = synapse lines [g; g*Esyn] from NonSpikingSynapse / SpikingSynapse / HybridSpikingSynapse (unconnected ports count as zero). Outputs: V [mV], spike event (0/1). Doctrine: Szczecinski et al. 2017/2020; sns_toolbox 1.5.2. The adaptive-threshold variant (threshold proportionality m, threshold increment) is future work.
      mask Display:
      | t_ = linspace(0, 2*pi, 73);
      | patch(0.95*cos(t_), 0.95*sin(t_), [0 0 0]);
      | patch(0.84*cos(t_), 0.84*sin(t_), [0.99 0.96 0.81]);
      | xs_ = [-0.58 -0.54 -0.50 -0.46 -0.36 -0.32 -0.28 -0.24 -0.14 -0.10 -0.06 -0.02 0.08 0.12 0.16 0.20 0.30 0.34 0.38 0.42 0.52 0.58];
      | ys_ = [-0.22 -0.22 0.40 -0.22 -0.22 -0.22 0.40 -0.22 -0.22 -0.22 0.40 -0.22 -0.22 -0.22 0.40 -0.22 -0.22 -0.22 0.40 -0.22 -0.22 -0.22];
      | color('black');
      | plot(xs_, ys_);
      | plot(xs_+0.012, ys_);
      | plot(xs_-0.012, ys_);
  SpikingSynapse : Subsystem  mask(SNS Spiking Synapse){gmax=1, ginc=1, tau_syn=20, Esyn=0}
      mask prompts: gmax "Max conductance gmax (uS)"; ginc "Conductance increment per spike (uS)"; tau_syn "Decay time constant tau_syn (ms)"; Esyn "Reversal potential Esyn (mV). >=0 excit, <0 inhib"
      mask help: Spiking chemical synapse, event-wired: input = the SPIKE output line of a SpikingNeuron / SpikingLIFNeuron. Conductance (sns_toolbox SpikingSynapse): exponential decay with tau_syn; on each presynaptic spike (rising edge) g <- min(gmax, g + ginc) — conductance_increment included, saturating at gmax. Output [g; g*Esyn] connects to ANY neuron's syn1..syn6 port (spiking or non-spiking postsynaptic cell). Esyn >= 0 excitatory (icon: white triangle), < 0 inhibitory (solid black circle).
      mask Display:
      | es_ = NaN;
      | try
      |     tmp_ = Esyn;
      |     if ischar(tmp_) || isstring(tmp_), tmp_ = eval(tmp_); end
      |     es_ = tmp_;
      | catch
      | end
      | if isnan(es_)
      |     patch([-1 1 1 -1], [-1 -1 1 1], [0.9 0.9 0.9]);
      |     disp('E?');
      | elseif es_ < 0
      |     patch([-1 1 1 -1], [-1 -1 1 1], [0.97 0.86 0.85]);
      |     patch([-1 0.58 0.58 -1], [0.42 0.42 0.58 0.58], [0 0 0]);
      |     t_ = linspace(0, 2*pi, 73);
      |     patch(0.18*cos(t_) + 0.72, 0.50*sin(t_), [0 0 0]);
      |     color('black');
      |     plot([-1 -0.75 -0.65 -0.55 -0.35 -0.25 -0.15 0.05 0.15 0.25 0.45 0.55 0.58], [0.50 0.50 0.72 0.50 0.50 0.72 0.50 0.50 0.72 0.50 0.50 0.50 0.50]);
      | else
      |     patch([-1 1 1 -1], [-1 -1 1 1], [0.85 0.94 0.86]);
      |     patch([-1 0.30 0.30 -1], [0.42 0.42 0.58 0.58], [0 0 0]);
      |     patch([0.30 0.90 0.90], [0.50 0.80 -0.20], [0 0 0]);
      |     patch([0.44 0.76 0.76], [0.50 0.70 -0.10], [1 1 1]);
      |     color('black');
      |     plot([-1 -0.75 -0.65 -0.55 -0.35 -0.25 -0.15 0.05 0.15 0.25 0.30], [0.50 0.50 0.72 0.50 0.50 0.72 0.50 0.50 0.72 0.50 0.50]);
      | end
  SynSum : Subsystem  mask(SNS Synapse Sum Junction){}
      mask help: Sums up to eight NonSpikingSynapse outputs ([g; g*Esyn] lines) into ONE synaptic signal for a NonSpikingNeuron syn port. Only needed when a neuron receives MORE than 6 synapses (the neuron has 6 syn ports): chain SynSum blocks for even more (a SynSum output can feed another SynSum input). Unconnected inputs count as zero.
      mask Display:
      | patch([-1 1 1 -1], [-1 -1 1 1], [0.93 0.93 0.93]);
      | color('black');
      | plot([-1 -0.1], [0.45 0.10]);
      | plot([-1 -0.1], [0.10 0.10]);
      | plot([-1 -0.1], [-0.45 0.10]);
      | plot([-0.1 1], [0.10 0.10]);
      | plot([-0.1 -0.1], [0.16 0.04]);

== system SNS_Library/BPAForce ==
  activation : Inport
  strain : Inport  Port=2
  Fmax_g : Gain  Gain=Fmax
  Fprod : Product
  Lterm : Sum  Inputs=+-
  Sat : Saturate  UpperLimit=Fmax  LowerLimit=0
  epsMax_c : Constant  Value=epsMax
  force_N : Outport
  wires:
  activation/1 -> Fmax_g/1
  epsMax_c/1 -> Lterm/1
  strain/1 -> Lterm/2
  Fmax_g/1 -> Fprod/1
  Lterm/1 -> Fprod/2
  Fprod/1 -> Sat/1
  Sat/1 -> force_N/1

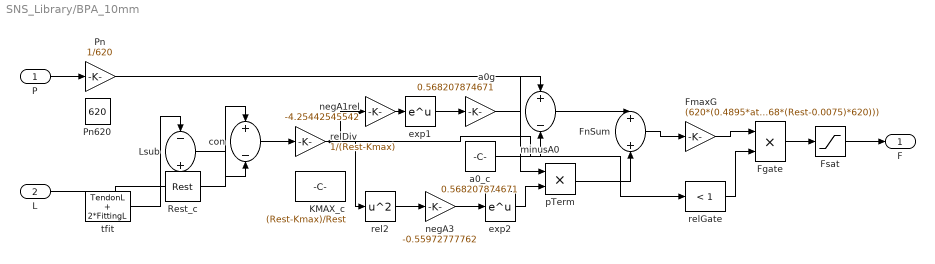
== system SNS_Library/BPA_10mm ==
  P : Inport
  L : Inport  Port=2
  Fgate : Product
  FmaxG : Gain  Gain=(620*(0.4895*atan(0.03068*(Rest-0.0075)*620)))
  FnSum : Sum
  Fsat : Saturate  UpperLimit=(620*(0.4895*atan(0.03068*(Rest-0.0075)*620)))  LowerLimit=0
  KMAX_c : Constant  Value=(Rest-Kmax)/Rest
  Lsub : Sum  Inputs=-+
  Pn : Gain  Gain=1/620
  Pn620 : Constant  Value=620
  Rest_c : Constant  Value=Rest
  a0_c : Constant  Value=0.568207874671
  a0g : Gain  Gain=0.568207874671
  con : Sum  Inputs=+-
  exp1 : Math
  exp2 : Math
  minusA0 : Sum  Inputs=+-
  negA1rel : Gain  Gain=-4.25442545542
  negA3 : Gain  Gain=-0.55972777762
  pTerm : Product
  rel2 : Math  Operator=square
  relDiv : Gain  Gain=1/(Rest-Kmax)
  relGate : simulink/Logic and Bit Operations/Compare To Constant  relop=<  const=1  OutDataTypeStr=boolean
  tfit : Constant  Value=TendonL + 2*FittingL
  F : Outport
  wires:
  P/1 -> Pn/1
  Pn/1 -> pTerm/1
  L/1 -> Lsub/2
  tfit/1 -> Lsub/1
  Lsub/1 -> con/2
  Rest_c/1 -> con/1
  con/1 -> relDiv/1
  relDiv/1 -> negA1rel/1, rel2/1, relGate/1
  negA1rel/1 -> exp1/1
  exp1/1 -> a0g/1
  a0g/1 -> minusA0/1
  a0_c/1 -> minusA0/2
  rel2/1 -> negA3/1
  negA3/1 -> exp2/1
  exp2/1 -> pTerm/2
  minusA0/1 -> FnSum/1
  pTerm/1 -> FnSum/2
  FnSum/1 -> FmaxG/1
  FmaxG/1 -> Fgate/1
  relGate/1 -> Fgate/2
  Fgate/1 -> Fsat/1
  Fsat/1 -> F/1

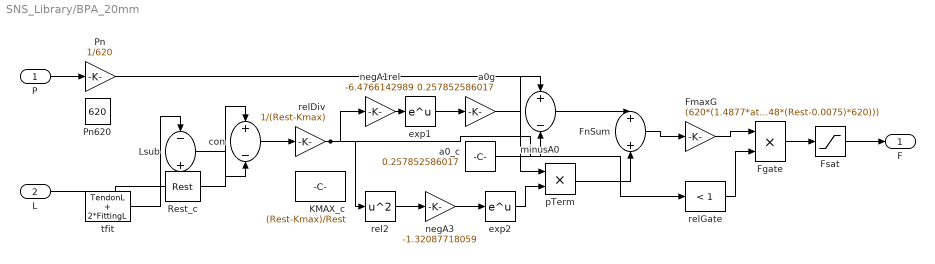
== system SNS_Library/BPA_20mm ==
  P : Inport
  L : Inport  Port=2
  Fgate : Product
  FmaxG : Gain  Gain=(620*(1.4877*atan(0.0248*(Rest-0.0075)*620)))
  FnSum : Sum
  Fsat : Saturate  UpperLimit=(620*(1.4877*atan(0.0248*(Rest-0.0075)*620)))  LowerLimit=0
  KMAX_c : Constant  Value=(Rest-Kmax)/Rest
  Lsub : Sum  Inputs=-+
  Pn : Gain  Gain=1/620
  Pn620 : Constant  Value=620
  Rest_c : Constant  Value=Rest
  a0_c : Constant  Value=0.257852586017
  a0g : Gain  Gain=0.257852586017
  con : Sum  Inputs=+-
  exp1 : Math
  exp2 : Math
  minusA0 : Sum  Inputs=+-
  negA1rel : Gain  Gain=-6.4766142989
  negA3 : Gain  Gain=-1.32087718059
  pTerm : Product
  rel2 : Math  Operator=square
  relDiv : Gain  Gain=1/(Rest-Kmax)
  relGate : simulink/Logic and Bit Operations/Compare To Constant  relop=<  const=1  OutDataTypeStr=boolean
  tfit : Constant  Value=TendonL + 2*FittingL
  F : Outport
  wires:
  P/1 -> Pn/1
  Pn/1 -> pTerm/1
  L/1 -> Lsub/2
  tfit/1 -> Lsub/1
  Lsub/1 -> con/2
  Rest_c/1 -> con/1
  con/1 -> relDiv/1
  relDiv/1 -> negA1rel/1, rel2/1, relGate/1
  negA1rel/1 -> exp1/1
  exp1/1 -> a0g/1
  a0g/1 -> minusA0/1
  a0_c/1 -> minusA0/2
  rel2/1 -> negA3/1
  negA3/1 -> exp2/1
  exp2/1 -> pTerm/2
  minusA0/1 -> FnSum/1
  pTerm/1 -> FnSum/2
  FnSum/1 -> FmaxG/1
  FmaxG/1 -> Fgate/1
  relGate/1 -> Fgate/2
  Fgate/1 -> Fsat/1
  Fsat/1 -> F/1

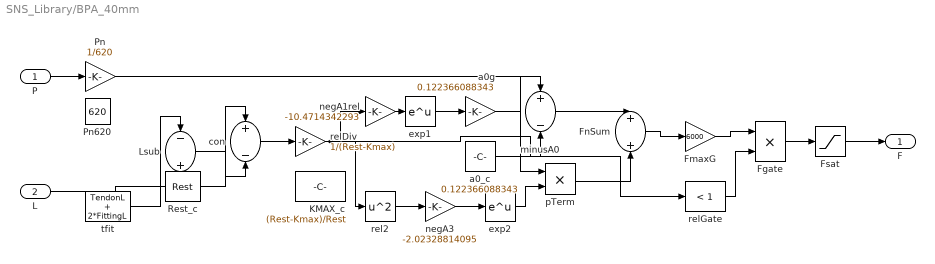
== system SNS_Library/BPA_40mm ==
  P : Inport
  L : Inport  Port=2
  Fgate : Product
  FmaxG : Gain  Gain=6000
  FnSum : Sum
  Fsat : Saturate  UpperLimit=6000  LowerLimit=0
  KMAX_c : Constant  Value=(Rest-Kmax)/Rest
  Lsub : Sum  Inputs=-+
  Pn : Gain  Gain=1/620
  Pn620 : Constant  Value=620
  Rest_c : Constant  Value=Rest
  a0_c : Constant  Value=0.122366088343
  a0g : Gain  Gain=0.122366088343
  con : Sum  Inputs=+-
  exp1 : Math
  exp2 : Math
  minusA0 : Sum  Inputs=+-
  negA1rel : Gain  Gain=-10.4714342293
  negA3 : Gain  Gain=-2.02328814095
  pTerm : Product
  rel2 : Math  Operator=square
  relDiv : Gain  Gain=1/(Rest-Kmax)
  relGate : simulink/Logic and Bit Operations/Compare To Constant  relop=<  const=1  OutDataTypeStr=boolean
  tfit : Constant  Value=TendonL + 2*FittingL
  F : Outport
  wires:
  P/1 -> Pn/1
  Pn/1 -> pTerm/1
  L/1 -> Lsub/2
  tfit/1 -> Lsub/1
  Lsub/1 -> con/2
  Rest_c/1 -> con/1
  con/1 -> relDiv/1
  relDiv/1 -> negA1rel/1, rel2/1, relGate/1
  negA1rel/1 -> exp1/1
  exp1/1 -> a0g/1
  a0g/1 -> minusA0/1
  a0_c/1 -> minusA0/2
  rel2/1 -> negA3/1
  negA3/1 -> exp2/1
  exp2/1 -> pTerm/2
  minusA0/1 -> FnSum/1
  pTerm/1 -> FnSum/2
  FnSum/1 -> FmaxG/1
  FmaxG/1 -> Fgate/1
  relGate/1 -> Fgate/2
  Fgate/1 -> Fsat/1
  Fsat/1 -> F/1

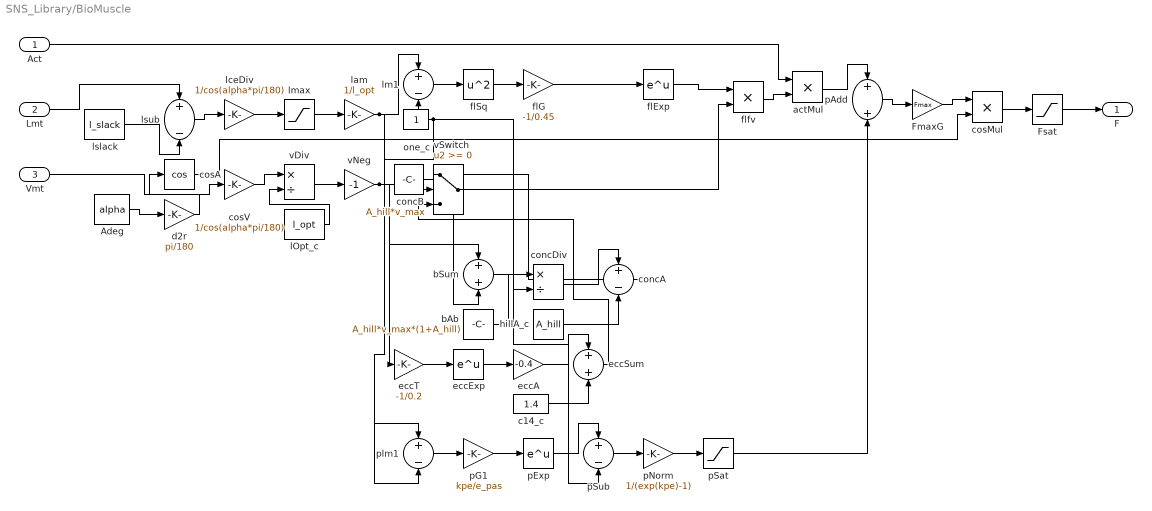
== system SNS_Library/BioMuscle ==
  Act : Inport
  Lmt : Inport  Port=2
  Vmt : Inport  Port=3
  Adeg : Constant  Value=alpha
  FmaxG : Gain  Gain=Fmax
  Fsat : Saturate  UpperLimit=2*Fmax  LowerLimit=0
  actMul : Product
  bAb : Constant  Value=A_hill*v_max*(1+A_hill)
  bSum : Sum
  c14_c : Constant  Value=1.4
  concA : Sum  Inputs=+-
  concB : Constant  Value=A_hill*v_max
  concDiv : Product  Inputs=*/
  cosA : Trigonometry  Operator=cos
  cosMul : Product
  cosV : Gain  Gain=1/cos(alpha*pi/180)
  d2r : Gain  Gain=pi/180
  eccA : Gain  Gain=-0.4
  eccExp : Math
  eccSum : Sum
  eccT : Gain  Gain=-1/0.2
  flExp : Math
  flG : Gain  Gain=-1/0.45
  flSq : Math  Operator=square
  flfv : Product
  hillA_c : Constant  Value=A_hill
  lOpt_c : Constant  Value=l_opt
  lam : Gain  Gain=1/l_opt
  lceDiv : Gain  Gain=1/cos(alpha*pi/180)
  lm1 : Sum  Inputs=+-
  lmax : Saturate  UpperLimit=10  LowerLimit=1e-3
  lslack : Constant  Value=l_slack
  lsub : Sum  Inputs=+-
  one_c : Constant
  pAdd : Sum
  pExp : Math
  pG1 : Gain  Gain=kpe/e_pas
  pNorm : Gain  Gain=1/(exp(kpe)-1)
  pSat : Saturate  UpperLimit=inf  LowerLimit=0
  pSub : Sum  Inputs=+-
  plm1 : Sum  Inputs=+-
  vDiv : Product  Inputs=*/
  vNeg : Gain  Gain=-1
  vSwitch : Switch  SaturateOnIntegerOverflow=off  InputSameDT=off
  F : Outport
  wires:
  Lmt/1 -> lsub/1
  lslack/1 -> lsub/2
  lsub/1 -> lceDiv/1
  lceDiv/1 -> lmax/1
  lmax/1 -> lam/1
  lam/1 -> lm1/1, plm1/1
  one_c/1 -> lm1/2, plm1/2, pSub/2
  lm1/1 -> flSq/1
  flSq/1 -> flG/1
  flG/1 -> flExp/1
  Adeg/1 -> d2r/1
  d2r/1 -> cosA/1
  Vmt/1 -> cosV/1
  cosV/1 -> vDiv/1
  lOpt_c/1 -> vDiv/2
  vDiv/1 -> vNeg/1
  vNeg/1 -> vSwitch/2, eccT/1, bSum/1
  concB/1 -> bSum/2
  bAb/1 -> concDiv/1
  bSum/1 -> concDiv/2
  concDiv/1 -> concA/1
  hillA_c/1 -> concA/2
  concA/1 -> vSwitch/1
  eccT/1 -> eccExp/1
  eccExp/1 -> eccA/1
  eccA/1 -> eccSum/1
  c14_c/1 -> eccSum/2
  eccSum/1 -> vSwitch/3
  plm1/1 -> pG1/1
  pG1/1 -> pExp/1
  pExp/1 -> pSub/1
  pSub/1 -> pNorm/1
  pNorm/1 -> pSat/1
  flExp/1 -> flfv/1
  vSwitch/1 -> flfv/2
  Act/1 -> actMul/1
  flfv/1 -> actMul/2
  actMul/1 -> pAdd/1
  pSat/1 -> pAdd/2
  pAdd/1 -> FmaxG/1
  FmaxG/1 -> cosMul/1
  cosA/1 -> cosMul/2
  cosMul/1 -> Fsat/1
  Fsat/1 -> F/1

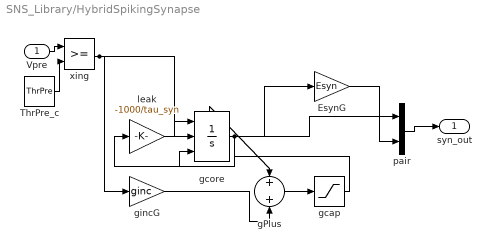
== system SNS_Library/HybridSpikingSynapse ==
  Vpre : Inport
  EsynG : Gain  Gain=Esyn
  ThrPre_c : Constant  Value=ThrPre
  gPlus : Sum
  gcap : Saturate  UpperLimit=gmax  LowerLimit=0
  gcore : Integrator  ExternalReset=rising  InitialConditionSource=external  ShowStatePort=on
  gincG : Gain  Gain=ginc  OutDataTypeStr=double
  leak : Gain  Gain=-1000/tau_syn
  pair : Mux  Inputs=2
  xing : RelationalOperator  OutDataTypeStr=boolean  RndMeth=Simplest  InputSameDT=off
  syn_out : Outport
  wires:
  Vpre/1 -> xing/1
  ThrPre_c/1 -> xing/2
  gcore/1 -> leak/1, EsynG/1, pair/1
  leak/1 -> gcore/1
  xing/1 -> gcore/2, gincG/1
  gcore/State -> gPlus/1
  gincG/1 -> gPlus/2
  gPlus/1 -> gcap/1
  gcap/1 -> gcore/3
  EsynG/1 -> pair/2
  pair/1 -> syn_out/1

== system SNS_Library/IaMuscleSpindle ==
  stretch : Inport
  vel : Inport  Port=2
  Sat : Saturate  UpperLimit=Imax  LowerLimit=0
  Wl_g : Gain  Gain=Wl
  Wv_g : Gain  Gain=Wv
  sumIa : Sum
  Isyn_nA : Outport
  wires:
  stretch/1 -> Wl_g/1
  vel/1 -> Wv_g/1
  Wl_g/1 -> sumIa/1
  Wv_g/1 -> sumIa/2
  sumIa/1 -> Sat/1
  Sat/1 -> Isyn_nA/1

== system SNS_Library/IbGolgiTendon ==
  force : Inport
  Kf_g : Gain  Gain=Kf
  Sat : Saturate  UpperLimit=Imax  LowerLimit=0
  Isyn_nA : Outport
  wires:
  force/1 -> Kf_g/1
  Kf_g/1 -> Sat/1
  Sat/1 -> Isyn_nA/1

== system SNS_Library/MuscleActivation ==
  S : Inport
  Aint : Integrator  InitialCondition=A0
  Sat : Saturate  UpperLimit=1  LowerLimit=0
  dA : Sum  Inputs=-+
  tauInv : Gain  Gain=1000/tauAct
  activation : Outport
  wires:
  S/1 -> dA/2
  Aint/1 -> dA/1, Sat/1
  dA/1 -> tauInv/1
  tauInv/1 -> Aint/1
  Sat/1 -> activation/1

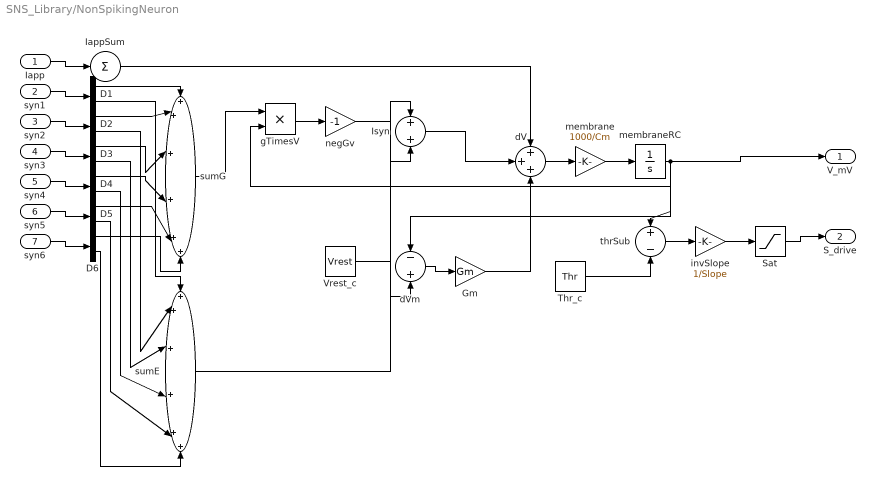
== system SNS_Library/NonSpikingNeuron ==
  Iapp : Inport
  syn1 : Inport  Port=2  PortDimensions=2
  syn2 : Inport  Port=3  PortDimensions=2
  syn3 : Inport  Port=4  PortDimensions=2
  syn4 : Inport  Port=5  PortDimensions=2
  syn5 : Inport  Port=6  PortDimensions=2
  syn6 : Inport  Port=7  PortDimensions=2
  D{1..6} (6 alike) : Demux  Outputs=2
  Gm : Gain  Gain=Gm
  IappSum : Sum  Inputs=+
  Isyn : Sum
  Sat : Saturate  UpperLimit=1  LowerLimit=0
  Thr_c : Constant  Value=Thr
  Vrest_c : Constant  Value=Vrest
  dV : Sum  Inputs=+++
  dVm : Sum  Inputs=-+
  gTimesV : Product
  invSlope : Gain  Gain=1/Slope
  membrane : Gain  Gain=1000/Cm
  membraneRC : Integrator  InitialCondition=Vrest
  negGv : Gain  Gain=-1
  sumE : Sum  Inputs=++++++
  sumG : Sum  Inputs=++++++
  thrSub : Sum  Inputs=+-
  V_mV : Outport
  S_drive : Outport  Port=2
  wires:
  syn1/1 -> D1/1
  D1/1 -> sumG/1
  D1/2 -> sumE/1
  syn2/1 -> D2/1
  D2/1 -> sumG/2
  D2/2 -> sumE/2
  syn3/1 -> D3/1
  D3/1 -> sumG/3
  D3/2 -> sumE/3
  syn4/1 -> D4/1
  D4/1 -> sumG/4
  D4/2 -> sumE/4
  syn5/1 -> D5/1
  D5/1 -> sumG/5
  D5/2 -> sumE/5
  syn6/1 -> D6/1
  D6/1 -> sumG/6
  D6/2 -> sumE/6
  Iapp/1 -> IappSum/1
  IappSum/1 -> dV/1
  sumG/1 -> gTimesV/1
  membraneRC/1 -> gTimesV/2, dVm/1, V_mV/1, thrSub/1
  gTimesV/1 -> negGv/1
  sumE/1 -> Isyn/1
  negGv/1 -> Isyn/2
  Isyn/1 -> dV/2
  Vrest_c/1 -> dVm/2
  dVm/1 -> Gm/1
  Gm/1 -> dV/3
  dV/1 -> membrane/1
  membrane/1 -> membraneRC/1
  Thr_c/1 -> thrSub/2
  thrSub/1 -> invSlope/1
  invSlope/1 -> Sat/1
  Sat/1 -> S_drive/1

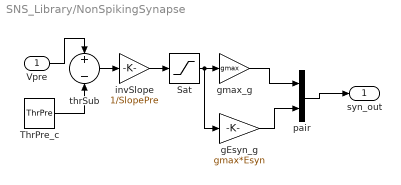
== system SNS_Library/NonSpikingSynapse ==
  Vpre : Inport
  Sat : Saturate  UpperLimit=1  LowerLimit=0
  ThrPre_c : Constant  Value=ThrPre
  gEsyn_g : Gain  Gain=gmax*Esyn
  gmax_g : Gain  Gain=gmax
  invSlope : Gain  Gain=1/SlopePre
  pair : Mux  Inputs=2
  thrSub : Sum  Inputs=+-
  syn_out : Outport
  wires:
  Vpre/1 -> thrSub/1
  ThrPre_c/1 -> thrSub/2
  thrSub/1 -> invSlope/1
  invSlope/1 -> Sat/1
  Sat/1 -> gmax_g/1, gEsyn_g/1
  gmax_g/1 -> pair/1
  gEsyn_g/1 -> pair/2
  pair/1 -> syn_out/1

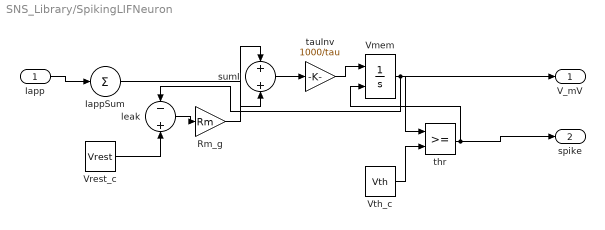
== system SNS_Library/SpikingLIFNeuron ==
  Iapp : Inport
  IappSum : Sum  Inputs=+
  Rm_g : Gain  Gain=Rm
  Vmem : Integrator  ExternalReset=rising  InitialCondition=Vrest
  Vrest_c : Constant  Value=Vrest
  Vth_c : Constant  Value=Vth
  leak : Sum  Inputs=-+
  sumI : Sum
  tauInv : Gain  Gain=1000/tau
  thr : RelationalOperator  OutDataTypeStr=boolean  RndMeth=Simplest  InputSameDT=off
  V_mV : Outport
  spike : Outport  Port=2
  wires:
  Iapp/1 -> IappSum/1
  IappSum/1 -> sumI/2
  Vrest_c/1 -> leak/2
  leak/1 -> Rm_g/1
  Rm_g/1 -> sumI/1
  sumI/1 -> tauInv/1
  tauInv/1 -> Vmem/1
  Vmem/1 -> leak/1, thr/1, V_mV/1
  Vth_c/1 -> thr/2
  thr/1 -> Vmem/2, spike/1

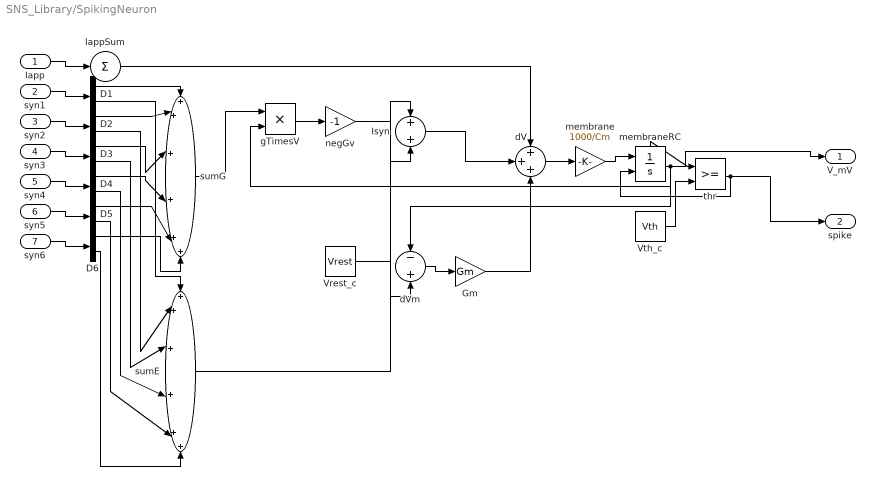
== system SNS_Library/SpikingNeuron ==
  Iapp : Inport
  syn1 : Inport  Port=2  PortDimensions=2
  syn2 : Inport  Port=3  PortDimensions=2
  syn3 : Inport  Port=4  PortDimensions=2
  syn4 : Inport  Port=5  PortDimensions=2
  syn5 : Inport  Port=6  PortDimensions=2
  syn6 : Inport  Port=7  PortDimensions=2
  D{1..6} (6 alike) : Demux  Outputs=2
  Gm : Gain  Gain=Gm
  IappSum : Sum  Inputs=+
  Isyn : Sum
  Vrest_c : Constant  Value=Vrest
  Vth_c : Constant  Value=Vth
  dV : Sum  Inputs=+++
  dVm : Sum  Inputs=-+
  gTimesV : Product
  membrane : Gain  Gain=1000/Cm
  membraneRC : Integrator  ExternalReset=rising  InitialCondition=Vreset  ShowStatePort=on
  negGv : Gain  Gain=-1
  sumE : Sum  Inputs=++++++
  sumG : Sum  Inputs=++++++
  thr : RelationalOperator  OutDataTypeStr=boolean  RndMeth=Simplest  InputSameDT=off
  V_mV : Outport
  spike : Outport  Port=2
  wires:
  syn1/1 -> D1/1
  D1/1 -> sumG/1
  D1/2 -> sumE/1
  syn2/1 -> D2/1
  D2/1 -> sumG/2
  D2/2 -> sumE/2
  syn3/1 -> D3/1
  D3/1 -> sumG/3
  D3/2 -> sumE/3
  syn4/1 -> D4/1
  D4/1 -> sumG/4
  D4/2 -> sumE/4
  syn5/1 -> D5/1
  D5/1 -> sumG/5
  D5/2 -> sumE/5
  syn6/1 -> D6/1
  D6/1 -> sumG/6
  D6/2 -> sumE/6
  Iapp/1 -> IappSum/1
  IappSum/1 -> dV/1
  sumG/1 -> gTimesV/1
  membraneRC/1 -> gTimesV/2, dVm/1, V_mV/1
  gTimesV/1 -> negGv/1
  sumE/1 -> Isyn/1
  negGv/1 -> Isyn/2
  Isyn/1 -> dV/2
  Vrest_c/1 -> dVm/2
  dVm/1 -> Gm/1
  Gm/1 -> dV/3
  dV/1 -> membrane/1
  membrane/1 -> membraneRC/1
  membraneRC/State -> thr/1
  Vth_c/1 -> thr/2
  thr/1 -> membraneRC/2, spike/1

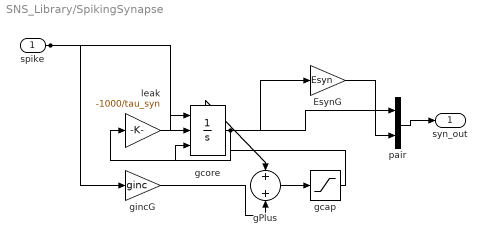
== system SNS_Library/SpikingSynapse ==
  spike : Inport
  EsynG : Gain  Gain=Esyn
  gPlus : Sum
  gcap : Saturate  UpperLimit=gmax  LowerLimit=0
  gcore : Integrator  ExternalReset=rising  InitialConditionSource=external  ShowStatePort=on
  gincG : Gain  Gain=ginc  OutDataTypeStr=double
  leak : Gain  Gain=-1000/tau_syn
  pair : Mux  Inputs=2
  syn_out : Outport
  wires:
  gcore/1 -> leak/1, EsynG/1, pair/1
  leak/1 -> gcore/1
  spike/1 -> gcore/2, gincG/1
  gcore/State -> gPlus/1
  gincG/1 -> gPlus/2
  gPlus/1 -> gcap/1
  gcap/1 -> gcore/3
  EsynG/1 -> pair/2
  pair/1 -> syn_out/1

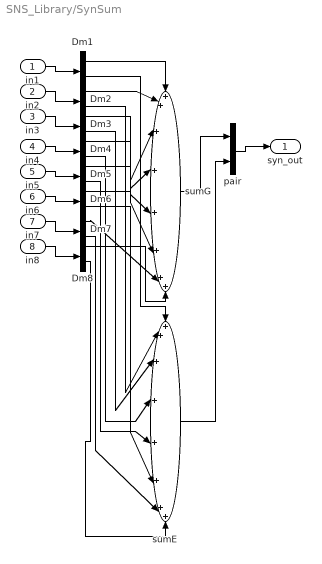
== system SNS_Library/SynSum ==
  in1 : Inport  PortDimensions=2
  in2 : Inport  Port=2  PortDimensions=2
  in3 : Inport  Port=3  PortDimensions=2
  in4 : Inport  Port=4  PortDimensions=2
  in5 : Inport  Port=5  PortDimensions=2
  in6 : Inport  Port=6  PortDimensions=2
  in7 : Inport  Port=7  PortDimensions=2
  in8 : Inport  Port=8  PortDimensions=2
  Dm{1..8} (8 alike) : Demux  Outputs=2
  pair : Mux  Inputs=2
  sumE : Sum  Inputs=++++++++
  sumG : Sum  Inputs=++++++++
  syn_out : Outport
  wires:
  in1/1 -> Dm1/1
  in2/1 -> Dm2/1
  in3/1 -> Dm3/1
  in4/1 -> Dm4/1
  in5/1 -> Dm5/1
  in6/1 -> Dm6/1
  in7/1 -> Dm7/1
  in8/1 -> Dm8/1
  Dm1/1 -> sumG/1
  Dm1/2 -> sumE/1
  Dm2/1 -> sumG/2
  Dm2/2 -> sumE/2
  Dm3/1 -> sumG/3
  Dm3/2 -> sumE/3
  Dm4/1 -> sumG/4
  Dm4/2 -> sumE/4
  Dm5/1 -> sumG/5
  Dm5/2 -> sumE/5
  Dm6/1 -> sumG/6
  Dm6/2 -> sumE/6
  Dm7/1 -> sumG/7
  Dm7/2 -> sumE/7
  Dm8/1 -> sumG/8
  Dm8/2 -> sumE/8
  sumG/1 -> pair/1
  sumE/1 -> pair/2
  pair/1 -> syn_out/1
